simulink model "acc_hil_plant"  (R2024b)
settings: Solver=ode1  StartTime=0.0  StopTime=60  FixedStep=0.05  RelTol=1e-3
settings Model: Creator=lukas  LastModifiedBy=lukas

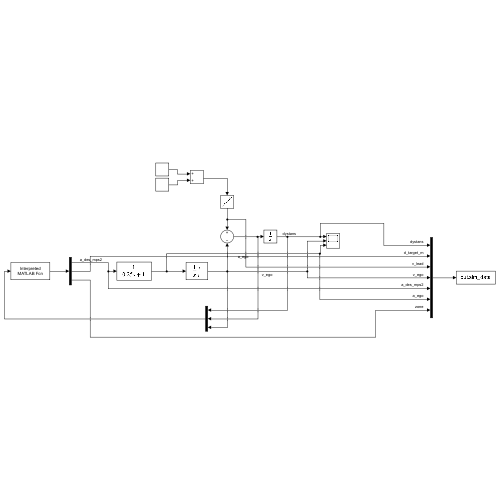
[thumbnail: Simulink's stored preview of the top-level diagram]
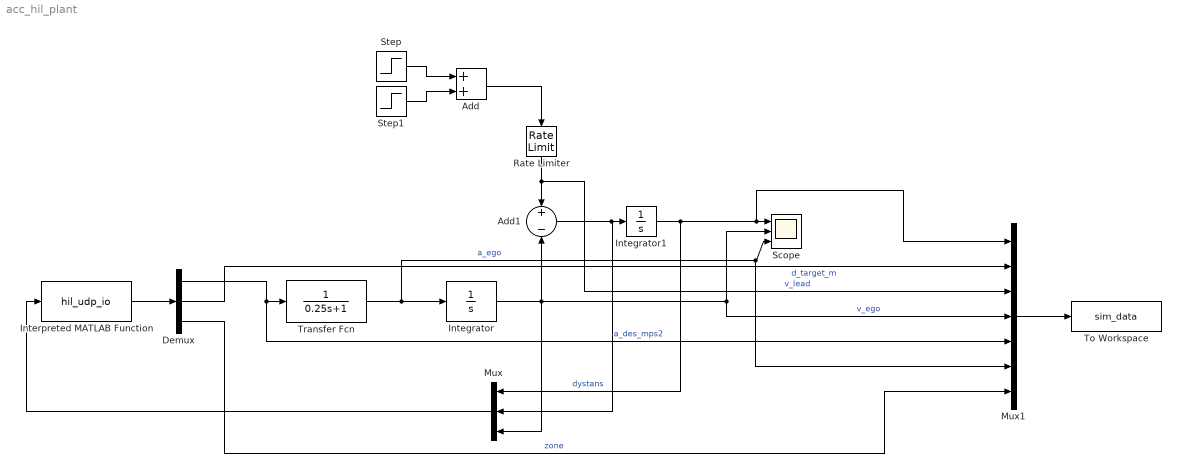
== system acc_hil_plant ==
  Add : Sum
  Add1 : Sum  Inputs=+-
  Demux : Demux  Outputs=3
  Integrator : Integrator  InitialCondition=20  LimitOutput=on  LowerSaturationLimit=0
  Integrator1 : Integrator  InitialCondition=60
  Interpreted MATLAB Function : MATLABFcn  MATLABFcn=hil_udp_io  OutputDimensions=3
  Mux : Mux  Inputs=3
  Mux1 : Mux  Inputs=7
  Rate Limiter : RateLimiter  RisingSlewLimit=1.5  FallingSlewLimit=-4.5  SampleTimeMode=inherited
  Scope : Scope  NumInputPorts=3
  Step : Step  Time=15  Before=20  After=0  SampleTime=0
  Step1 : Step  Time=35  After=15  SampleTime=0
  To Workspace : ToWorkspace  VariableName=sim_data  SampleTime=0.05
  Transfer Fcn : TransferFcn  Denominator=[0.25 1]
  wires:
  Add1/1 -> Mux/2, Integrator1/1
  Transfer Fcn/1 -> Integrator/1, Mux1/6, Scope/3  "a_ego"
  Integrator/1 -> Add1/2, Mux/3, Scope/2, Mux1/4  "v_ego"
  Mux/1 -> Interpreted MATLAB Function/1
  Integrator1/1 -> Mux1/1, Scope/1, Mux/1  "dystans"
  Interpreted MATLAB Function/1 -> Demux/1
  Demux/1 -> Transfer Fcn/1, Mux1/5  "a_des_mps2"
  Step/1 -> Add/1
  Step1/1 -> Add/2
  Rate Limiter/1 -> Mux1/3, Add1/1  "v_lead"
  Add/1 -> Rate Limiter/1
  Demux/2 -> Mux1/2  "d_target_m"
  Mux1/1 -> To Workspace/1
  Demux/3 -> Mux1/7  "zone"
